simulink model "estimation_velocity"  (R2024b)
settings: configuration reference "MCConfiguration" (kept outside this file)
model workspace (MAT data in the model file):
  EstimationVelocity_Ts = Simulink.Parameter
  EstimationVelocity_Ts.Value = 0.001
  EstimationVelocity_Ts.Complexity = 'real'
  EstimationVelocity_Ts.Dimensions = [1 1]
  EstimationVelocity_Ts.DataType = 'auto'
  EstimationVelocity_Ts.DocUnits = 's'
libraries: dspbuff3 x1, dsppolyfun x1
settings Model: DataDictionary=embeddedBoard_common.sldd  Creator=ascalzo  LastModifiedBy=mfussi
settings ConfigSetRef: SourceName=MCConfiguration

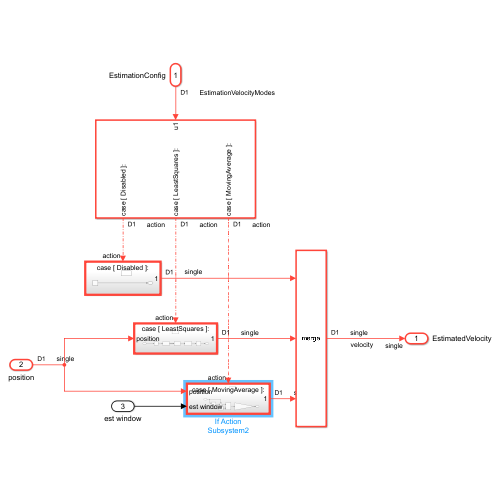
[thumbnail: Simulink's stored preview of the top-level diagram]
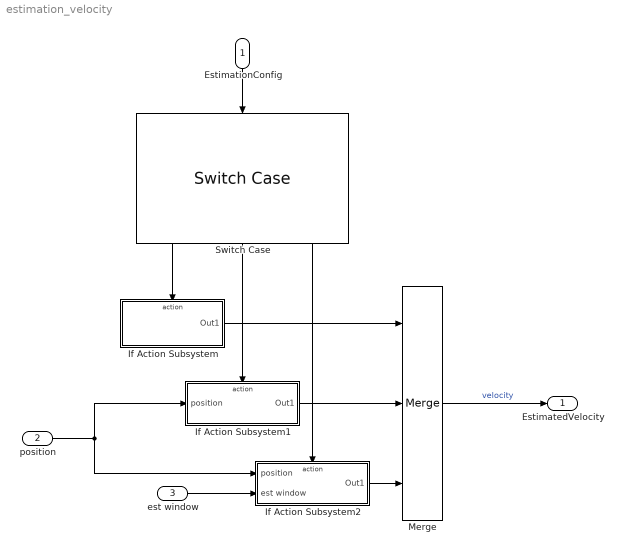
== system estimation_velocity ==
  EstimationConfig : Inport  OutDataTypeStr=Enum: EstimationVelocityModes  BusOutputAsStruct=on
  position : Inport  Port=2  OutDataTypeStr=single
  est window : Inport  Port=3
  If Action Subsystem : Subsystem  TreatAsAtomicUnit=on
  If Action Subsystem1 : Subsystem  TreatAsAtomicUnit=on
  If Action Subsystem2 : Subsystem  TreatAsAtomicUnit=on
  Merge : Merge  Inputs=3
  Switch Case : SwitchCase  CaseConditions={EstimationVelocityModes.Disabled,EstimationVelocityModes.LeastSquares,EstimationVelocityModes.MovingAverage}  ShowDefaultCase=off
  EstimatedVelocity : Outport  OutDataTypeStr=single  Unit=deg/s  LockScale=on  BusOutputAsStruct=on
  wires:
  position/1 -> If Action Subsystem1/1(position), If Action Subsystem2/1(position)
  Merge/1 -> EstimatedVelocity/1  "velocity"
  EstimationConfig/1 -> Switch Case/1
  Switch Case/1 -> If Action Subsystem/Action
  Switch Case/2 -> If Action Subsystem1/Action
  Switch Case/3 -> If Action Subsystem2/Action
  If Action Subsystem/1(Out1) -> Merge/1
  If Action Subsystem1/1(Out1) -> Merge/2
  If Action Subsystem2/1(Out1) -> Merge/3
  est window/1 -> If Action Subsystem2/2(est window)

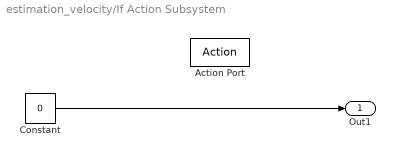
== system estimation_velocity/If Action Subsystem ==
  Action Port : ActionPort  ActionPortLabel=case [ Disabled ]:
  Constant : Constant  Value=0  OutDataTypeStr=single  SampleTime=-1
  Out1 : Outport
  wires:
  Constant/1 -> Out1/1

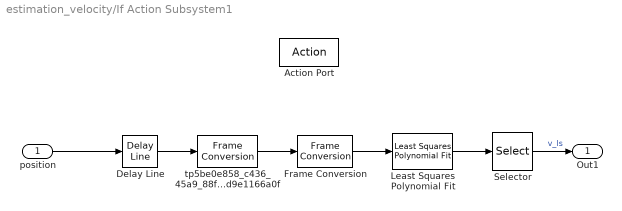
== system estimation_velocity/If Action Subsystem1 ==
  position : Inport
  Action Port : ActionPort  ActionPortLabel=case [ LeastSquares ]:
  Delay Line : dspbuff3/Delay Line  siz=16  ic=0  directfeed=on  enable_output=off  hold_output=off  OutputFrames=off
  Frame Conversion : FrameConversion  OutFrame=Sample-based
  Least Squares Polynomial Fit : dsppolyfun/Least Squares Polynomial Fit  X=(0:15) * EstimationVelocity_Ts  N=1
  Selector : Selector  InputPortWidth=2  IndexOptions=Index vector (dialog)  Indices=1  OutputSizes=1
  tp5be0e858_c436_45a9_88fb_67d9e1166a0f : FrameConversion
  Out1 : Outport
  wires:
  tp5be0e858_c436_45a9_88fb_67d9e1166a0f/1 -> Frame Conversion/1
  Delay Line/1 -> tp5be0e858_c436_45a9_88fb_67d9e1166a0f/1
  Frame Conversion/1 -> Least Squares Polynomial Fit/1
  Least Squares Polynomial Fit/1 -> Selector/1
  Selector/1 -> Out1/1  "v_ls"
  position/1 -> Delay Line/1

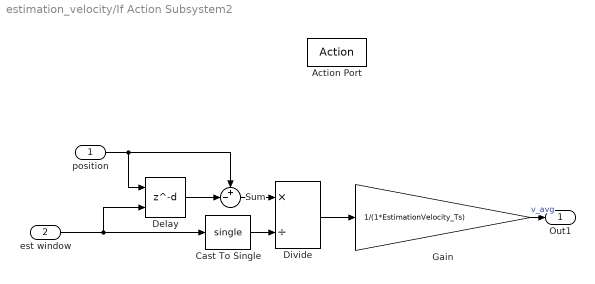
== system estimation_velocity/If Action Subsystem2 ==
  position : Inport
  est window : Inport  Port=2
  Action Port : ActionPort  ActionPortLabel=case [ MovingAverage ]:
  Cast To Single : DataTypeConversion  OutDataTypeStr=single  SaturateOnIntegerOverflow=off  RndMeth=Floor
  Delay : Delay  DelayLengthSource=Input port  DelayLength=64  UseCircularBuffer=on
      settings: InputPortMap=u0,p1
  Divide : Product  Inputs=*/
  Gain : Gain  Gain=1/(1*EstimationVelocity_Ts)
  Sum : Sum  Inputs=+-|
  Out1 : Outport
  wires:
  Gain/1 -> Out1/1  "v_avg"
  position/1 -> Delay/1, Sum/1
  Delay/1 -> Sum/2
  Sum/1 -> Divide/1
  Divide/1 -> Gain/1
  est window/1 -> Delay/2, Cast To Single/1
  Cast To Single/1 -> Divide/2
